simulink model "PV_SYSTEM_WITH_VARIOUS_MPPT"  (R2017a)
settings: Solver=ode45  StartTime=0.0  StopTime=2  RelTol=1e-3  EnableMultiTasking=on
undefined symbols (not defined in the file): dEgdT, EgRef, gcbh, k1, Rsh_array5pc, sigbuilder_block, sps_rtmsupport, Tref_K, Ts, VT_ref
libraries: powerlib x16, neural x15, simulink x4, spsPVarrayModel x3, powerlib_extras x2, fuzblock x1, powerlib_meascontrol x1
(part 6 of 6)

== system PV_SYSTEM_WITH_VARIOUS_MPPT/MATLAB//SIMULINK  BLOCK/      ==
  In1 : Inport
  In2 : Inport  Port=2
  Gain : Gain  Gain=100
  div1 : Product  Inputs=/*  RndMeth=Zero
  Out1 : Outport
  wires:
  Gain/1 -> Out1/1
  div1/1 -> Gain/1
  In2/1 -> div1/2
  In1/1 -> div1/1

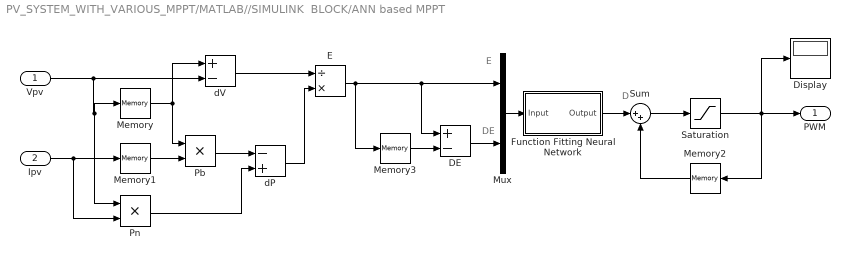
== system PV_SYSTEM_WITH_VARIOUS_MPPT/MATLAB//SIMULINK  BLOCK/ANN based MPPT ==
  note: E
  note: DE
  note: D
  Vpv : Inport
  Ipv : Inport  Port=2
  DE : Sum  Inputs=+-
  Display : Display
  E : Product  Inputs=/*
  Function Fitting Neural Network : Subsystem
      mask help: Function Fitting Neural Network
      mask Display: e = 0.06;c1 = [120 150 230]/255;c2 = ([120 150 230]+0)/383;c3 = ([120 150 230]+128)/383;patch([0 1 1 0],[0 0 1 1],c1);patch([0 1 1 1-e 1-e 0+e],[0 0 1 1-e 0+e 0+e],c2);patch([0 0 1 1-e 0+e 0+e],[0 1 1 1-e 1-e 0+e],c3);plot([0 1 1 0 0],[0 0 1 1 0]);fprintf('NNET');port_label('input',1,' Input');port_label('output',1,'Output ');
  Memory{,1..3} (4 alike) : Memory  InheritSampleTime=on
  Mux : Mux  Inputs=2
  Pb : Product
  Pn : Product
  Saturation : Saturate  UpperLimit=0.9  LowerLimit=0.1
  Sum : Sum  Inputs=|++
  dP : Sum  Inputs=-+
  dV : Sum  Inputs=+-
  PWM : Outport
  wires:
  Function Fitting Neural Network/1(Output) -> Sum/1
  Mux/1 -> Function Fitting Neural Network/1(Input)
  Sum/1 -> Saturation/1
  dV/1 -> E/1
  E/1 -> Memory3/1, Mux/1, DE/1
  dP/1 -> E/2
  Vpv/1 -> dV/2, Memory/1, Pn/1
  Saturation/1 -> Memory2/1, PWM/1, Display/1
  DE/1 -> Mux/2
  Memory3/1 -> DE/2
  Memory2/1 -> Sum/2
  Pn/1 -> dP/2
  Pb/1 -> dP/1
  Memory1/1 -> Pb/2
  Ipv/1 -> Memory1/1, Pn/2
  Memory/1 -> dV/1, Pb/1

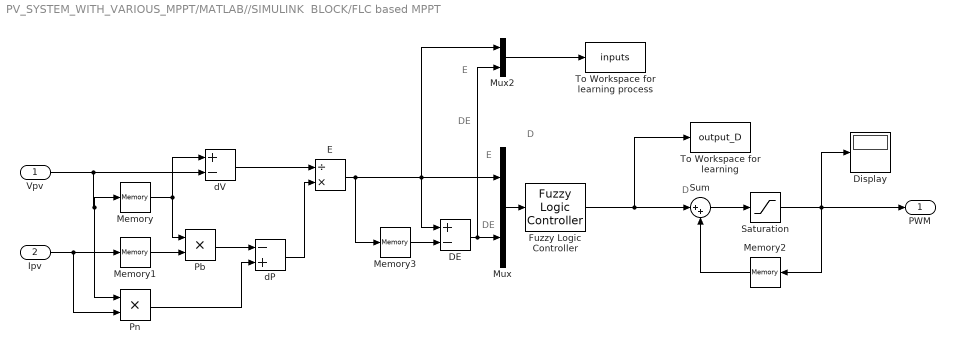
== system PV_SYSTEM_WITH_VARIOUS_MPPT/MATLAB//SIMULINK  BLOCK/FLC based MPPT ==
  note: DE
  note: D
  note: E
  note: D
  note: DE
  note: E
  Vpv : Inport
  Ipv : Inport  Port=2
  DE : Sum  Inputs=+-
  Display : Display
  E : Product  Inputs=/*
  Fuzzy Logic Controller : fuzblock/Fuzzy Logic  Controller  fis=mppt
  Memory{,1..3} (4 alike) : Memory  InheritSampleTime=on
  Mux : Mux  Inputs=2
  Mux2 : Mux  Inputs=2
  Pb : Product
  Pn : Product
  Saturation : Saturate  UpperLimit=0.9  LowerLimit=0.1
  Sum : Sum  Inputs=|++
  To Workspace for learning : ToWorkspace  VariableName=output_D  SampleTime=1e-6
      settings: MaxDataPoints=10000  Save2DSignal=2-D array (concatenate along first dimension)
  To Workspace for learning process : ToWorkspace  VariableName=inputs  SampleTime=1e-6
      settings: MaxDataPoints=100000  Save2DSignal=2-D array (concatenate along first dimension)
  dP : Sum  Inputs=-+
  dV : Sum  Inputs=+-
  PWM : Outport
  wires:
  Memory/1 -> Pb/1, dV/1
  Ipv/1 -> Pn/2, Memory1/1
  Memory1/1 -> Pb/2
  Pb/1 -> dP/1
  Pn/1 -> dP/2
  Memory2/1 -> Sum/2
  Memory3/1 -> DE/2
  DE/1 -> Mux/2, Mux2/2
  Saturation/1 -> Display/1, PWM/1, Memory2/1
  Vpv/1 -> Pn/1, Memory/1, dV/2
  dP/1 -> E/2
  E/1 -> DE/1, Mux/1, Mux2/1, Memory3/1
  dV/1 -> E/1
  Sum/1 -> Saturation/1
  Mux/1 -> Fuzzy Logic Controller/1
  Mux2/1 -> To Workspace for learning process/1
  Fuzzy Logic Controller/1 -> To Workspace for learning/1, Sum/1

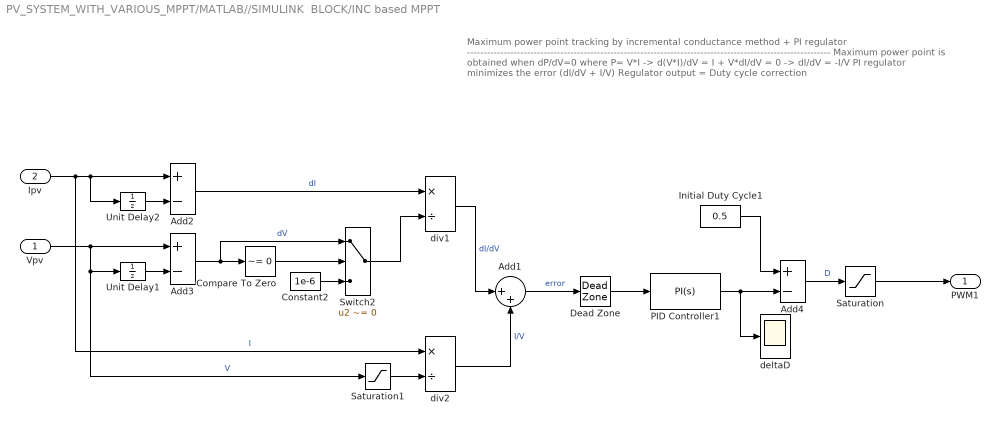
== system PV_SYSTEM_WITH_VARIOUS_MPPT/MATLAB//SIMULINK  BLOCK/INC based MPPT ==
  note: Maximum power point tracking by incremental conductance method + PI regulator
      | -------------------------------------------------------------------------------------------------------------
      | Maximum power point is obtained when dP/dV=0  where P= V*I
      | -> d(V*I)/dV = I + V*dI/dV = 0
      | -> dI/dV = -I/V
      | PI regulator minimizes the error (dI/dV + I/V)
      | Regulator output = Duty cycle correction
  Vpv : Inport
  Ipv : Inport  Port=2
  Add1 : Sum  Inputs=|++
  Add2 : Sum  Inputs=+-
  Add3 : Sum  Inputs=+-
  Add4 : Sum  Inputs=+-
  Compare To Zero : simulink/Logic and Bit Operations/Compare To Zero  relop=~=  OutDataTypeStr=uint8
  Constant2 : Constant  Value=1e-6
  Dead Zone : DeadZone  LowerValue=-0.02  UpperValue=+0.02  SaturateOnIntegerOverflow=on
  Initial Duty Cycle1 : Constant  Value=0.5
  PID Controller1 : simulink/Continuous/PID Controller  Controller=PI  TimeDomain=Continuous-time  SampleTime=-1  IntegratorMethod=Forward Euler  FilterMethod=Forward Euler  Form=Parallel  UseFilter=on  ControllerParametersSource=internal  P=8  I=20  D=0  N=100  InitialConditionSource=internal  InitialConditionForIntegrator=0  InitialConditionForFilter=0  ExternalReset=none  LimitOutput=on  UpperSaturationLimit=1  LowerSaturationLimit=-1  LinearizeAsGain=on  AntiWindupMode=none  Kb=1  TrackingMode=off  Kt=1  PParamMin=[]  PParamMax=[]  IParamMin=[]  IParamMax=[]  DParamMin=[]  DParamMax=[]  NParamMin=[]  NParamMax=[]  KbParamMin=[]  KbParamMax=[]  KtParamMin=[]  KtParamMax=[]  POutMin=[]  POutMax=[]  IOutMin=[]  IOutMax=[]  DOutMin=[]  DOutMax=[]  NOutMin=[]  NOutMax=[]  KbOutMin=[]  KbOutMax=[]  KtOutMin=[]  KtOutMax=[]  IntegratorOutMin=[]  IntegratorOutMax=[]  FilterOutMin=[]  FilterOutMax=[]  SumOutMin=[]  SumOutMax=[]  SumI1OutMin=[]  SumI1OutMax=[]  SumI2OutMin=[]  SumI2OutMax=[]  SumI3OutMin=[]  SumI3OutMax=[]  SumDOutMin=[]  SumDOutMax=[]  SaturationOutMin=[]  SaturationOutMax=[]  IntegratorContinuousStateAttributes=''  IntegratorStateMustResolveToSignalObject=off  IntegratorRTWStateStorageClass=Auto  FilterContinuousStateAttributes=''  FilterStateMustResolveToSignalObject=off  FilterRTWStateStorageClass=Auto  DifferentiatorICPrevScaledInput=0  DifferentiatorOutMin=[]  DifferentiatorOutMax=[]  InitialConditionSetting=State (most efficient)
  Saturation : Saturate  UpperLimit=1  LowerLimit=0
  Saturation1 : Saturate  UpperLimit=inf  LowerLimit=eps
  Switch2 : Switch  Criteria=u2 ~= 0
  Unit Delay1 : UnitDelay  SampleTime=Ts
  Unit Delay2 : UnitDelay  SampleTime=Ts
  deltaD : Scope
  div1 : Product  Inputs=*/  RndMeth=Zero
  div2 : Product  Inputs=*/  RndMeth=Zero
  PWM1 : Outport
  wires:
  Add4/1 -> Saturation/1  "D"
  PID Controller1/1 -> deltaD/1, Add4/2
  Initial Duty Cycle1/1 -> Add4/1
  Add3/1 -> Compare To Zero/1, Switch2/1  "dV"
  div2/1 -> Add1/2  "I/V"
  Saturation1/1 -> div2/2
  Unit Delay1/1 -> Add3/2
  Add2/1 -> div1/1  "dI"
  Switch2/1 -> div1/2
  Unit Delay2/1 -> Add2/2
  Ipv/1 -> Unit Delay2/1, Add2/1, div2/1  "I"
  div1/1 -> Add1/1  "dI/dV"
  Compare To Zero/1 -> Switch2/2
  Constant2/1 -> Switch2/3
  Vpv/1 -> Add3/1, Saturation1/1, Unit Delay1/1  "V"
  Add1/1 -> Dead Zone/1  "error"
  Dead Zone/1 -> PID Controller1/1
  Saturation/1 -> PWM1/1

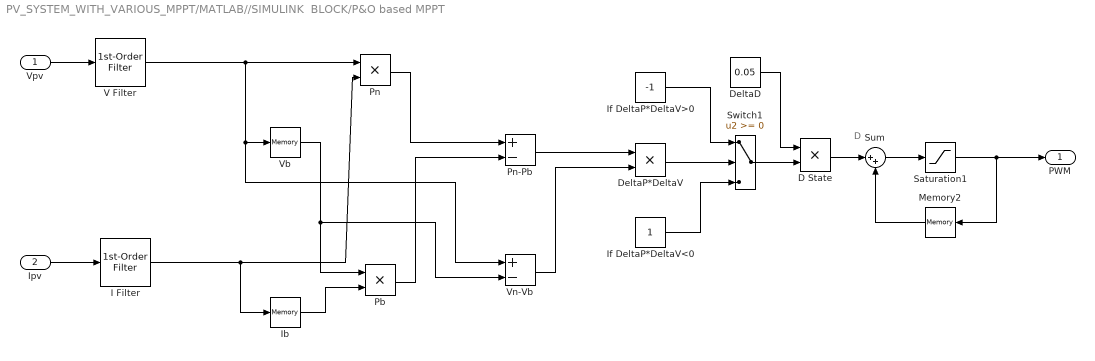
== system PV_SYSTEM_WITH_VARIOUS_MPPT/MATLAB//SIMULINK  BLOCK/P&O based MPPT ==
  note: D
  Vpv : Inport
  Ipv : Inport  Port=2
  D State : Product  RndMeth=Zero
  DeltaD : Constant  Value=0.05
  DeltaP*DeltaV : Product  RndMeth=Zero
  I Filter : powerlib_extras/Control  Blocks/1st-Order  Filter  FilterType=Lowpass  Tc=1e-3  Initialize=off  Vac_Init=[0.8 -25 60]  Vdc_Init=-0.4  PlotResponse=off  param1=[1 500 1]
  Ib : Memory  InheritSampleTime=on  LinearizeAsDelay=on
  If DeltaP*DeltaV<0 : Constant
  If DeltaP*DeltaV>0 : Constant  Value=-1
  Memory2 : Memory  InheritSampleTime=on
  Pb : Product  RndMeth=Zero
  Pn : Product  RndMeth=Zero
  Pn-Pb : Sum  Inputs=+-
  Saturation1 : Saturate  UpperLimit=0.9  LowerLimit=0.1
  Sum : Sum  Inputs=|++
  Switch1 : Switch
  V Filter : powerlib_extras/Control  Blocks/1st-Order  Filter  FilterType=Lowpass  Tc=1e-3  Initialize=off  Vac_Init=[0.8 -25 60]  Vdc_Init=-0.4  PlotResponse=off  param1=[1 500 1]
  Vb : Memory  InheritSampleTime=on  LinearizeAsDelay=on
  Vn-Vb : Sum  Inputs=+-
  PWM : Outport
  wires:
  Ipv/1 -> I Filter/1
  If DeltaP*DeltaV<0/1 -> Switch1/3
  Pn/1 -> Pn-Pb/1
  V Filter/1 -> Vn-Vb/1, Vb/1, Pn/1
  Ib/1 -> Pb/2
  DeltaP*DeltaV/1 -> Switch1/2
  Vb/1 -> Vn-Vb/2, Pb/1
  If DeltaP*DeltaV>0/1 -> Switch1/1
  Pn-Pb/1 -> DeltaP*DeltaV/1
  Vn-Vb/1 -> DeltaP*DeltaV/2
  I Filter/1 -> Pn/2, Ib/1
  Vpv/1 -> V Filter/1
  Pb/1 -> Pn-Pb/2
  Switch1/1 -> D State/2
  DeltaD/1 -> D State/1
  D State/1 -> Sum/1
  Sum/1 -> Saturation1/1
  Memory2/1 -> Sum/2
  Saturation1/1 -> PWM/1, Memory2/1

== system PV_SYSTEM_WITH_VARIOUS_MPPT/MATLAB//SIMULINK  BLOCK/X-Y Plotter ==
  x : Inport
  y : Inport  Port=2
  Setting : Constant  Value=[N xmin xmax ymin ymax]
  X-Y Animated Plotter : MATLAB Function  TreatAsAtomicUnit=on  SystemSampleTime=tsam
  wires:
  Setting/1 -> X-Y Animated Plotter/3(set)
  y/1 -> X-Y Animated Plotter/2(y)
  x/1 -> X-Y Animated Plotter/1(x)

== system PV_SYSTEM_WITH_VARIOUS_MPPT/MATLAB//SIMULINK  BLOCK/	PV panels of LREA laboratory /Irradiance  ==
  Demux : Demux  Tag=STV Demux  Outputs=2
  FromWs : FromWorkspace  Tag=STV FromWs  VariableName=tuvar  SampleTime=0
      SigBuilderData=|
      | common.afterFinalStr = 'Extrapolate'
      | common.sampleTime = '0'
      | dataSet(1).timeRange = [0 2]
      | dataSet(1).name = 'Constant Irradiance'
      | dataSet(2).timeRange = [0 2]
      | dataSet(2).name = 'Step Irradiance'
      | dataSet(3).timeRange = [0 1]
      | dataSet(3).name = 'Ramp-up/down Irradiance'
      | sbobj.Groups(1).Name = 'Constant Irradiance'
      | sbobj.Groups(1).Signals(1).Name = 'Ir'
      | sbobj.Groups(1).Signals(1).XData = [0 2]
      | sbobj.Groups(1).Signals(1).YData = [1000 1000]
      | sbobj.Groups(1).Signals(2).Name = 'Temp'
      | sbobj.Groups(1).Signals(2).XData = [0 1 1 2]
      | sbobj.Groups(1).Signals(2).YData = [0 0 1 1]
      | sbobj.Groups(1).TimeRange = [0 2]
      | sbobj.Groups(2).Name = 'Step Irradiance'
      | sbobj.Groups(2).Signals(1).Name = 'Ir'
      | sbobj.Groups(2).Signals(1).XData = [0 0.252 0.252 2]
      | sbobj.Groups(2).Signals(1).YData = [600 600 1000 1000]
      | sbobj.Groups(2).Signals(2).Name = 'Temp'
      | sbobj.Groups(2).Signals(2).XData = [0 1 1 2]
      | sbobj.Groups(2).Signals(2).YData = [0 0 1 1]
      | sbobj.Groups(2).TimeRange = [0 2]
      | sbobj.Groups(3).Name = 'Ramp-up/down Irradiance'
      | sbobj.Groups(3).Signals(1).Name = 'Ir'
      | sbobj.Groups(3).Signals(1).XData = [0 0.3 0.3 0.4 0.4 0.5 0.5 1]
      | sbobj.Groups(3).Signals(1).YData = [1000 1000 800 795 600 600 400 395]
      | sbobj.Groups(3).Signals(2).Name = 'Temp'
      | sbobj.Groups(3).Signals(2).XData = [0 1]
      | sbobj.Groups(3).Signals(2).YData = [25 25]
      | sbobj.Groups(3).TimeRange = [0 1]
  Ir : Outport  Tag=STV Outport
  Temp : Outport  Tag=STV Outport  Port=2
  wires:
  Demux/1 -> Ir/1
  FromWs/1 -> Demux/1
  Demux/2 -> Temp/1

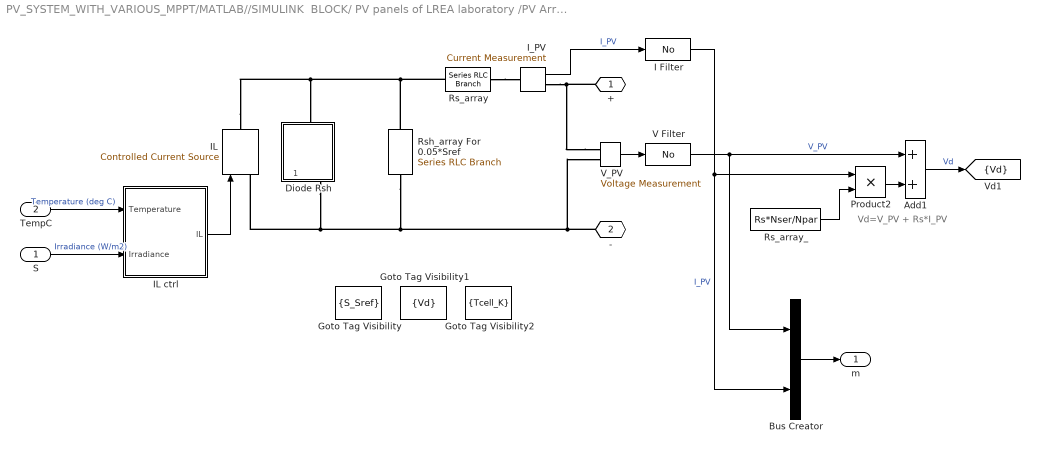
== system PV_SYSTEM_WITH_VARIOUS_MPPT/MATLAB//SIMULINK  BLOCK/	PV panels of LREA laboratory /PV Array ==
  note: Vd=V_PV + Rs*I_PV
  S : Inport
  TempC : Inport  Port=2
  Add1 : Sum
  Bus Creator : BusCreator  Inputs=2
  Diode Rsh : Subsystem
      mask Display:
      | plot(-75,-50,100,150, [-15 -15 43 -15 -15 -75],[50 8 50 92 50 50], ...
      |     [43 43],[8 94],[100 43], [50 50])
  Goto Tag Visibility : GotoTagVisibility  GotoTag=S_Sref
  Goto Tag Visibility1 : GotoTagVisibility  GotoTag=Vd
  Goto Tag Visibility2 : GotoTagVisibility  GotoTag=Tcell_K
  I Filter : spsPVarrayModel/No  VariantControl=Variant1
  IL : powerlib/Electrical Sources/Controlled Current Source  Initialize=on  Source_Type=AC  Amplitude=0  Phase=0  Frequency=0  Measurements=None
  IL ctrl : Subsystem
  I_PV : powerlib/Measurements/Current Measurement  PhasorSimulation=off  OutputType=Complex  PSBequivalent=0
  Product2 : Product  Inputs=**  RndMeth=Zero
  Rs_array : powerlib/Elements/Series RLC Branch  LConnTagsString=__new0  RConnTagsString=__new0  BranchType=R  Resistance=Rs*Nser/Npar  Inductance=1e-3  SetiL0=off  InitialCurrent=0  Capacitance=1e-6  Setx0=off  InitialVoltage=0  Measurements=None
  Rs_array_ : Constant  Value=Rs*Nser/Npar
  Rsh_array For 0.05*Sref : powerlib/Elements/Series RLC Branch  LConnTagsString=__new0  RConnTagsString=__new0  BranchType=R  Resistance=Rsh_array5pc  Inductance=1e-3  SetiL0=off  InitialCurrent=0  Capacitance=1e-6  Setx0=off  InitialVoltage=0  Measurements=None
  V Filter : spsPVarrayModel/No  VariantControl=Variant1
  V_PV : powerlib/Measurements/Voltage Measurement  PhasorSimulation=off  OutputType=Complex  PSBequivalent=0
  + : PMIOPort  Port=1  Side=Right
  - : PMIOPort  Port=2  Side=Right
  m : Outport
  tag scope: Vd=scoped
  wires:
  V Filter/1 -> Add1/1, Bus Creator/1  "V_PV"
  I Filter/1 -> Product2/1, Bus Creator/2  "I_PV"
  V_PV/1 -> V Filter/1
  IL ctrl/1(IL) -> IL/1
  Bus Creator/1 -> m/1
  Rs_array_/1 -> Product2/2
  Product2/1 -> Add1/2
  I_PV/1 -> I Filter/1  "I_PV"
  Add1/1 -> [Vd]  "Vd"
  S/1 -> IL ctrl/2(Irradiance)  "Irradiance (W/m2)"
  TempC/1 -> IL ctrl/1(Temperature)  "Temperature (deg C)"
  connections:
  Rs_array/RConn1 -- I_PV/LConn1
  IL/LConn1 -- Diode Rsh/RConn1 -- Rsh_array For 0.05*Sref/RConn1 -- -/RConn1 -- V_PV/LConn2
  IL/RConn1 -- Rsh_array For 0.05*Sref/LConn1 -- Rs_array/LConn1 -- Diode Rsh/LConn1
  V_PV/LConn1 -- I_PV/RConn1 -- +/RConn1

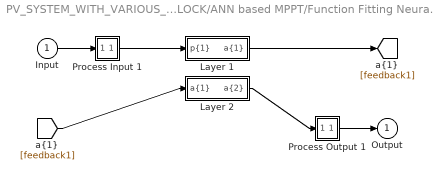
== system PV_SYSTEM_WITH_VARIOUS_MPPT/MATLAB//SIMULINK  BLOCK/ANN based MPPT/Function Fitting Neural Network ==
  Input : Inport  PortDimensions=2
      mask Display: e = 0.06;c1 = [120 230 180]/255;c2 = ([120 230 180]+0)/(256+128);c3 = ([120 230 180]+128)/(256+128);patch([0 1 1 0],[0 0 1 1],c1);patch([0 1 1 1-e 1-e 0+e],[0 0 1 1-e 0+e 0+e],c2);patch([0 0 1 1-e 0+e 0+e],[0 1 1 1-e 1-e 0+e],c3);plot([0 1 1 0 0],[0 0 1 1 0]);
  Layer 1 : Subsystem
      mask Display: e = 0.06;c1 = [120 150 230]/255;c2 = ([120 150 230]+0)/383;c3 = ([120 150 230]+128)/383;patch([0 1 1 0],[0 0 1 1],c1);patch([0 1 1 1-e 1-e 0+e],[0 0 1 1-e 0+e 0+e],c2);patch([0 0 1 1-e 0+e 0+e],[0 1 1 1-e 1-e 0+e],c3);plot([0 1 1 0 0],[0 0 1 1 0]);
  Layer 2 : Subsystem
      mask Display: e = 0.06;c1 = [120 150 230]/255;c2 = ([120 150 230]+0)/383;c3 = ([120 150 230]+128)/383;patch([0 1 1 0],[0 0 1 1],c1);patch([0 1 1 1-e 1-e 0+e],[0 0 1 1-e 0+e 0+e],c2);patch([0 0 1 1-e 0+e 0+e],[0 1 1 1-e 1-e 0+e],c3);plot([0 1 1 0 0],[0 0 1 1 0]);
  Process Input 1 : Subsystem
      mask Display: e = 0.06;c1 = [120 150 230]/255;c2 = ([120 150 230]+0)/383;c3 = ([120 150 230]+128)/383;patch([0 1 1 0],[0 0 1 1],c1);patch([0 1 1 1-e 1-e 0+e],[0 0 1 1-e 0+e 0+e],c2);patch([0 0 1 1-e 0+e 0+e],[0 1 1 1-e 1-e 0+e],c3);plot([0 1 1 0 0],[0 0 1 1 0]);
  Process Output 1 : Subsystem
      mask Display: e = 0.06;c1 = [120 150 230]/255;c2 = ([120 150 230]+0)/383;c3 = ([120 150 230]+128)/383;patch([0 1 1 0],[0 0 1 1],c1);patch([0 1 1 1-e 1-e 0+e],[0 0 1 1-e 0+e 0+e],c2);patch([0 0 1 1-e 0+e 0+e],[0 1 1 1-e 1-e 0+e],c3);plot([0 1 1 0 0],[0 0 1 1 0]);
  Output : Outport  InitialOutput=0
      mask Display: e = 0.06;c1 = [120 230 180]/255;c2 = ([120 230 180]+0)/(256+128);c3 = ([120 230 180]+128)/(256+128);patch([0 1 1 0],[0 0 1 1],c1);patch([0 1 1 1-e 1-e 0+e],[0 0 1 1-e 0+e 0+e],c2);patch([0 0 1 1-e 0+e 0+e],[0 1 1 1-e 1-e 0+e],c3);plot([0 1 1 0 0],[0 0 1 1 0]);
  wires:
  Layer 2/1("a{2}") -> Process Output 1/1(a)
  [feedback1] -> Layer 2/1("a{1} ")
  Layer 1/1("a{1}") -> [feedback1]
  Process Input 1/1(p) -> Layer 1/1("p{1}")
  Process Output 1/1(y) -> Output/1
  Input/1 -> Process Input 1/1(x)

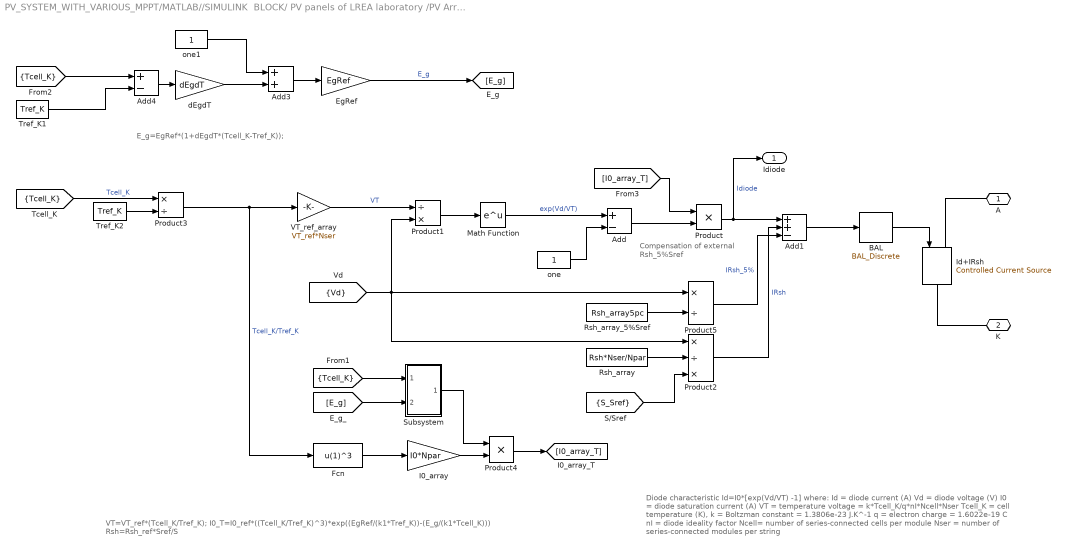
== system PV_SYSTEM_WITH_VARIOUS_MPPT/MATLAB//SIMULINK  BLOCK/	PV panels of LREA laboratory /PV Array/Diode Rsh ==
  note: Compensation of
      | external Rsh_5%Sref
  note: Diode characteristic
      |    Id=I0*[exp(Vd/VT) -1]
      |
      | where:
      |      Id = diode current (A)
      |      Vd = diode voltage (V)
      |      I0 = diode saturation current (A)
      |      VT = temperature voltage = k*Tcell_K/q*nI*Ncell*Nser
      | Tcell_K = cell temperature (K),
      |       k = Boltzman constant = 1.3806e-23 J.K^-1
      |       q = electron charge = 1.6022e-19 C
      |      nI = diode ideality factor
      |    Ncell= number of series-connected cells per module
      |    Nser = number of series-connected modules per string
  note: VT=VT_ref*(Tcell_K/Tref_K);
      | I0_T=I0_ref*((Tcell_K/Tref_K)^3)*exp((EgRef/(k1*Tref_K))-(E_g/(k1*Tcell_K)))
      | Rsh=Rsh_ref*Sref/S
  note: E_g=EgRef*(1+dEgdT*(Tcell_K-Tref_K));
  Add : Sum  Inputs=+-
  Add1 : Sum  Inputs=++-
  Add3 : Sum
  Add4 : Sum  Inputs=+-
  BAL : spsPVarrayModel/BAL_Discrete  VariantControl=NoBAL
  EgRef : Gain  Gain=EgRef
  Fcn : Fcn  Expr=u(1)^3
  I0_array : Gain  Gain=I0*Npar
  Id+IRsh : powerlib/Electrical Sources/Controlled Current Source  Initialize=on  Source_Type=AC  Amplitude=0  Phase=0  Frequency=0  Measurements=None
  Math Function : Math  SaturateOnIntegerOverflow=on
  Product : Product  RndMeth=Zero
  Product1 : Product  Inputs=/*  RndMeth=Zero
  Product2 : Product  Inputs=*/*  RndMeth=Zero
  Product3 : Product  Inputs=*/  RndMeth=Zero
  Product4 : Product  Inputs=**  RndMeth=Zero
  Product5 : Product  Inputs=*/  RndMeth=Zero
  Rsh_array : Constant  Value=Rsh*Nser/Npar
  Rsh_array_5%Sref : Constant  Value=Rsh_array5pc
  Subsystem : Subsystem
  Tref_K1 : Constant  Value=Tref_K
  Tref_K2 : Constant  Value=Tref_K
  VT_ref_array : Gain  Gain=VT_ref*Nser
  dEgdT : Gain  Gain=dEgdT
  one : Constant
  one1 : Constant
  A : PMIOPort  Port=1  Side=Left
  K : PMIOPort  Port=2  Side=Right
  Idiode : Outport
  wires:
  BAL/1 -> Id+IRsh/1
  Add1/1 -> BAL/1
  Product5/1 -> Add1/3  "IRsh_5%"
  Rsh_array_5%Sref/1 -> Product5/2
  Math Function/1 -> Add/1  "exp(Vd/VT)"
  Product2/1 -> Add1/2  "IRsh"
  Product/1 -> Add1/1, Idiode/1  "Idiode"
  Product1/1 -> Math Function/1
  one/1 -> Add/2
  Rsh_array/1 -> Product2/2
  [Tcell_K] -> Product3/1  "Tcell_K"
  Product3/1 -> VT_ref_array/1, Fcn/1  "Tcell_K/Tref_K"
  one1/1 -> Add3/1
  Add4/1 -> dEgdT/1
  dEgdT/1 -> Add3/2
  Add3/1 -> EgRef/1
  EgRef/1 -> [E_g]  "E_g"
  I0_array/1 -> Product4/2
  Fcn/1 -> I0_array/1
  [Tcell_K] -> Add4/1
  Tref_K1/1 -> Add4/2
  Subsystem/1(exp) -> Product4/1
  [Tcell_K] -> Subsystem/1(Tcell_K)
  [E_g] -> Subsystem/2(E_g)
  Tref_K2/1 -> Product3/2
  Product4/1 -> [I0_array_T]
  Add/1 -> Product/2
  VT_ref_array/1 -> Product1/1  "VT"
  [I0_array_T] -> Product/1
  [S_Sref] -> Product2/3
  [Vd] -> Product5/1, Product2/1, Product1/2
  connections:
  Id+IRsh/RConn1 -- K/RConn1
  A/RConn1 -- Id+IRsh/LConn1

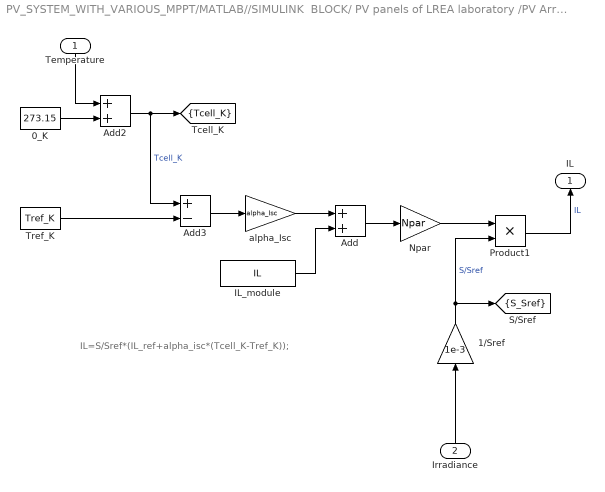
== system PV_SYSTEM_WITH_VARIOUS_MPPT/MATLAB//SIMULINK  BLOCK/	PV panels of LREA laboratory /PV Array/IL ctrl ==
  note: IL=S/Sref*(IL_ref+alpha_isc*(Tcell_K-Tref_K));
  Temperature : Inport
  Irradiance : Inport  Port=2
  0_K : Constant  Value=273.15
  1/Sref : Gain  Gain=1e-3
  Add : Sum
  Add2 : Sum
  Add3 : Sum  Inputs=+-
  IL_module : Constant  Value=IL
  Npar : Gain  Gain=Npar
  Product1 : Product  Inputs=**  RndMeth=Zero
  Tref_K : Constant  Value=Tref_K
  alpha_Isc : Gain  Gain=alpha_Isc
  IL : Outport
  tag scope: S_Sref=scoped, Tcell_K=scoped
  wires:
  Temperature/1 -> Add2/1
  Irradiance/1 -> 1/Sref/1
  alpha_Isc/1 -> Add/1
  Add3/1 -> alpha_Isc/1
  Tref_K/1 -> Add3/2
  Product1/1 -> IL/1  "IL"
  IL_module/1 -> Add/2
  0_K/1 -> Add2/2
  Add/1 -> Npar/1
  Add2/1 -> Add3/1, [Tcell_K]  "Tcell_K"
  Npar/1 -> Product1/1
  1/Sref/1 -> Product1/2, [S_Sref]  "S/Sref"

== system PV_SYSTEM_WITH_VARIOUS_MPPT/MATLAB//SIMULINK  BLOCK/ANN based MPPT/Function Fitting Neural Network/Layer 1 ==
  "p{1}" : Inport  PortDimensions=2
      mask Display: e = 0.06;c1 = [120 230 180]/255;c2 = ([120 230 180]+0)/(256+128);c3 = ([120 230 180]+128)/(256+128);patch([0 1 1 0],[0 0 1 1],c1);patch([0 1 1 1-e 1-e 0+e],[0 0 1 1-e 0+e 0+e],c2);patch([0 0 1 1-e 0+e 0+e],[0 1 1 1-e 1-e 0+e],c3);plot([0 1 1 0 0],[0 0 1 1 0]);
  Delays 1 : Subsystem
      mask Display: e = 0.06;c1 = [120 150 230]/255;c2 = ([120 150 230]+0)/383;c3 = ([120 150 230]+128)/383;patch([0 1 1 0],[0 0 1 1],c1);patch([0 1 1 1-e 1-e 0+e],[0 0 1 1-e 0+e 0+e],c2);patch([0 0 1 1-e 0+e 0+e],[0 1 1 1-e 1-e 0+e],c3);plot([0 1 1 0 0],[0 0 1 1 0]);disp('0');
  "IW{1,1}" : Subsystem
      mask Display: e = 0.06;c1 = [120 150 230]/255;c2 = ([120 150 230]+0)/383;c3 = ([120 150 230]+128)/383;patch([0 1 1 0],[0 0 1 1],c1);patch([0 1 1 1-e 1-e 0+e],[0 0 1 1-e 0+e 0+e],c2);patch([0 0 1 1-e 0+e 0+e],[0 1 1 1-e 1-e 0+e],c3);plot([0 1 1 0 0],[0 0 1 1 0]);disp('W');
  "b{1}" : Constant  Value=[4.2498450600033646;-3.5459947004323884;-2.8437309415280434;1.9169166361344252;-0.42994895301969316;-0.41524374608432507;1.5012029363474229;2.4596143283853529;3.4420068184056949;4.4215289791863901]
      mask Display: e = 0.06;c1 = [120 150 230]/255;c2 = ([120 150 230]+0)/383;c3 = ([120 150 230]+128)/383;patch([0 1 1 0],[0 0 1 1],c1);patch([0 1 1 1-e 1-e 0+e],[0 0 1 1-e 0+e 0+e],c2);patch([0 0 1 1-e 0+e 0+e],[0 1 1 1-e 1-e 0+e],c3);plot([0 1 1 0 0],[0 0 1 1 0]);disp('b');
  netsum : Sum  Inputs=2  SaturateOnIntegerOverflow=on  InputSameDT=on  OutDataTypeStr=Inherit: Same as first input
      mask Display: e = 0.06;c1 = [120 150 230]/255;c2 = ([120 150 230]+0)/383;c3 = ([120 150 230]+128)/383;patch([0 1 1 0],[0 0 1 1],c1);patch([0 1 1 1-e 1-e 0+e],[0 0 1 1-e 0+e 0+e],c2);patch([0 0 1 1-e 0+e 0+e],[0 1 1 1-e 1-e 0+e],c3);plot([0 1 1 0 0],[0 0 1 1 0]);disp('+');
  tansig : neural/Transfer Functions/tansig
  "a{1}" : Outport  InitialOutput=[0;0;0;0;0;0;0;0;0;0]
      mask Display: e = 0.06;c1 = [120 230 180]/255;c2 = ([120 230 180]+0)/(256+128);c3 = ([120 230 180]+128)/(256+128);patch([0 1 1 0],[0 0 1 1],c1);patch([0 1 1 1-e 1-e 0+e],[0 0 1 1-e 0+e 0+e],c2);patch([0 0 1 1-e 0+e 0+e],[0 1 1 1-e 1-e 0+e],c3);plot([0 1 1 0 0],[0 0 1 1 0]);
  wires:
  tansig/1 -> "a{1}"/1
  netsum/1 -> tansig/1
  "b{1}"/1 -> netsum/2
  "IW{1,1}"/1("iz{1,1}") -> netsum/1
  Delays 1/1("pd{1,1}") -> "IW{1,1}"/1("pd{1,1}")
  "p{1}"/1 -> Delays 1/1("p{1}")

== system PV_SYSTEM_WITH_VARIOUS_MPPT/MATLAB//SIMULINK  BLOCK/ANN based MPPT/Function Fitting Neural Network/Layer 2 ==
  "a{1} " : Inport  PortDimensions=10
      mask Display: e = 0.06;c1 = [120 230 180]/255;c2 = ([120 230 180]+0)/(256+128);c3 = ([120 230 180]+128)/(256+128);patch([0 1 1 0],[0 0 1 1],c1);patch([0 1 1 1-e 1-e 0+e],[0 0 1 1-e 0+e 0+e],c2);patch([0 0 1 1-e 0+e 0+e],[0 1 1 1-e 1-e 0+e],c3);plot([0 1 1 0 0],[0 0 1 1 0]);
  Delays 1 : Subsystem
      mask Display: e = 0.06;c1 = [120 150 230]/255;c2 = ([120 150 230]+0)/383;c3 = ([120 150 230]+128)/383;patch([0 1 1 0],[0 0 1 1],c1);patch([0 1 1 1-e 1-e 0+e],[0 0 1 1-e 0+e 0+e],c2);patch([0 0 1 1-e 0+e 0+e],[0 1 1 1-e 1-e 0+e],c3);plot([0 1 1 0 0],[0 0 1 1 0]);disp('0');
  "LW{2,1}" : Subsystem
      mask Display: e = 0.06;c1 = [120 150 230]/255;c2 = ([120 150 230]+0)/383;c3 = ([120 150 230]+128)/383;patch([0 1 1 0],[0 0 1 1],c1);patch([0 1 1 1-e 1-e 0+e],[0 0 1 1-e 0+e 0+e],c2);patch([0 0 1 1-e 0+e 0+e],[0 1 1 1-e 1-e 0+e],c3);plot([0 1 1 0 0],[0 0 1 1 0]);disp('W');
  "b{2}" : Constant  Value=1.5159961723017756
      mask Display: e = 0.06;c1 = [120 150 230]/255;c2 = ([120 150 230]+0)/383;c3 = ([120 150 230]+128)/383;patch([0 1 1 0],[0 0 1 1],c1);patch([0 1 1 1-e 1-e 0+e],[0 0 1 1-e 0+e 0+e],c2);patch([0 0 1 1-e 0+e 0+e],[0 1 1 1-e 1-e 0+e],c3);plot([0 1 1 0 0],[0 0 1 1 0]);disp('b');
  netsum : Sum  Inputs=2  SaturateOnIntegerOverflow=on  InputSameDT=on  OutDataTypeStr=Inherit: Same as first input
      mask Display: e = 0.06;c1 = [120 150 230]/255;c2 = ([120 150 230]+0)/383;c3 = ([120 150 230]+128)/383;patch([0 1 1 0],[0 0 1 1],c1);patch([0 1 1 1-e 1-e 0+e],[0 0 1 1-e 0+e 0+e],c2);patch([0 0 1 1-e 0+e 0+e],[0 1 1 1-e 1-e 0+e],c3);plot([0 1 1 0 0],[0 0 1 1 0]);disp('+');
  purelin : neural/Transfer Functions/purelin
  "a{2}" : Outport  InitialOutput=0
      mask Display: e = 0.06;c1 = [120 230 180]/255;c2 = ([120 230 180]+0)/(256+128);c3 = ([120 230 180]+128)/(256+128);patch([0 1 1 0],[0 0 1 1],c1);patch([0 1 1 1-e 1-e 0+e],[0 0 1 1-e 0+e 0+e],c2);patch([0 0 1 1-e 0+e 0+e],[0 1 1 1-e 1-e 0+e],c3);plot([0 1 1 0 0],[0 0 1 1 0]);
  wires:
  purelin/1 -> "a{2}"/1
  netsum/1 -> purelin/1
  "b{2}"/1 -> netsum/2
  "LW{2,1}"/1("lz{2,1}") -> netsum/1
  Delays 1/1("pd{2,1}") -> "LW{2,1}"/1("ad{2,1}")
  "a{1} "/1 -> Delays 1/1("p{2}")

== system PV_SYSTEM_WITH_VARIOUS_MPPT/MATLAB//SIMULINK  BLOCK/ANN based MPPT/Function Fitting Neural Network/Process Input 1 ==
  x : Inport  PortDimensions=2
      mask Display: e = 0.06;c1 = [120 230 180]/255;c2 = ([120 230 180]+0)/(256+128);c3 = ([120 230 180]+128)/(256+128);patch([0 1 1 0],[0 0 1 1],c1);patch([0 1 1 1-e 1-e 0+e],[0 0 1 1-e 0+e 0+e],c2);patch([0 0 1 1-e 0+e 0+e],[0 1 1 1-e 1-e 0+e],c3);plot([0 1 1 0 0],[0 0 1 1 0]);
  mapminmax : neural/Processing Functions/mapminmax  xmin=[-94.016320043316156;-101.91504684015196]  xmax=[7.8987267968357999;90.85267225948256]  ymin=-1  ymax=1
  p : Outport  PortDimensions=2
      mask Display: e = 0.06;c1 = [120 230 180]/255;c2 = ([120 230 180]+0)/(256+128);c3 = ([120 230 180]+128)/(256+128);patch([0 1 1 0],[0 0 1 1],c1);patch([0 1 1 1-e 1-e 0+e],[0 0 1 1-e 0+e 0+e],c2);patch([0 0 1 1-e 0+e 0+e],[0 1 1 1-e 1-e 0+e],c3);plot([0 1 1 0 0],[0 0 1 1 0]);
  wires:
  mapminmax/1 -> p/1
  x/1 -> mapminmax/1

== system PV_SYSTEM_WITH_VARIOUS_MPPT/MATLAB//SIMULINK  BLOCK/ANN based MPPT/Function Fitting Neural Network/Process Output 1 ==
  a : Inport  PortDimensions=1
      mask Display: e = 0.06;c1 = [120 230 180]/255;c2 = ([120 230 180]+0)/(256+128);c3 = ([120 230 180]+128)/(256+128);patch([0 1 1 0],[0 0 1 1],c1);patch([0 1 1 1-e 1-e 0+e],[0 0 1 1-e 0+e 0+e],c2);patch([0 0 1 1-e 0+e 0+e],[0 1 1 1-e 1-e 0+e],c3);plot([0 1 1 0 0],[0 0 1 1 0]);
  mapminmax_reverse : neural/Processing Functions/mapminmax_reverse  xmin=-0.033148830521161396  xmax=0.087011804847006088  ymin=-1  ymax=1
  y : Outport  PortDimensions=1
      mask Display: e = 0.06;c1 = [120 230 180]/255;c2 = ([120 230 180]+0)/(256+128);c3 = ([120 230 180]+128)/(256+128);patch([0 1 1 0],[0 0 1 1],c1);patch([0 1 1 1-e 1-e 0+e],[0 0 1 1-e 0+e 0+e],c2);patch([0 0 1 1-e 0+e 0+e],[0 1 1 1-e 1-e 0+e],c3);plot([0 1 1 0 0],[0 0 1 1 0]);
  wires:
  mapminmax_reverse/1 -> y/1
  a/1 -> mapminmax_reverse/1

== system PV_SYSTEM_WITH_VARIOUS_MPPT/MATLAB//SIMULINK  BLOCK/	PV panels of LREA laboratory /PV Array/Diode Rsh/Subsystem ==
  note: exp((EgRef/(k1*Tref_K))-(E_g/(k1*Tcell_K)))
  Tcell_K : Inport
  E_g : Inport  Port=2
  Add : Sum  Inputs=+-
  EgRef : Constant  Value=EgRef/(k1*Tref_K)
  Math Function : Math  SaturateOnIntegerOverflow=on
  Product : Product  Inputs=*/
  k1 : Gain  Gain=k1
  exp : Outport
  wires:
  EgRef/1 -> Add/1
  E_g/1 -> Product/1
  Tcell_K/1 -> k1/1
  k1/1 -> Product/2
  Product/1 -> Add/2
  Add/1 -> Math Function/1
  Math Function/1 -> exp/1

== system PV_SYSTEM_WITH_VARIOUS_MPPT/MATLAB//SIMULINK  BLOCK/ANN based MPPT/Function Fitting Neural Network/Layer 1/Delays 1 ==
  "p{1}" : Inport  PortDimensions=2
      mask Display: e = 0.06;c1 = [120 230 180]/255;c2 = ([120 230 180]+0)/(256+128);c3 = ([120 230 180]+128)/(256+128);patch([0 1 1 0],[0 0 1 1],c1);patch([0 1 1 1-e 1-e 0+e],[0 0 1 1-e 0+e 0+e],c2);patch([0 0 1 1-e 0+e 0+e],[0 1 1 1-e 1-e 0+e],c3);plot([0 1 1 0 0],[0 0 1 1 0]);
  mux : Mux  Inputs=1
      mask Display: e = 0.06;c1 = [120 150 230]/255;c2 = ([120 150 230]+0)/383;c3 = ([120 150 230]+128)/383;patch([0 1 1 0],[0 0 1 1],c1);patch([0 1 1 1-e 1-e 0+e],[0 0 1 1-e 0+e 0+e],c2);patch([0 0 1 1-e 0+e 0+e],[0 1 1 1-e 1-e 0+e],c3);plot([0 1 1 0 0],[0 0 1 1 0]);disp('Mux')
  "pd{1,1}" : Outport
      mask Display: e = 0.06;c1 = [120 230 180]/255;c2 = ([120 230 180]+0)/(256+128);c3 = ([120 230 180]+128)/(256+128);patch([0 1 1 0],[0 0 1 1],c1);patch([0 1 1 1-e 1-e 0+e],[0 0 1 1-e 0+e 0+e],c2);patch([0 0 1 1-e 0+e 0+e],[0 1 1 1-e 1-e 0+e],c3);plot([0 1 1 0 0],[0 0 1 1 0]);
  wires:
  mux/1 -> "pd{1,1}"/1
  "p{1}"/1 -> mux/1

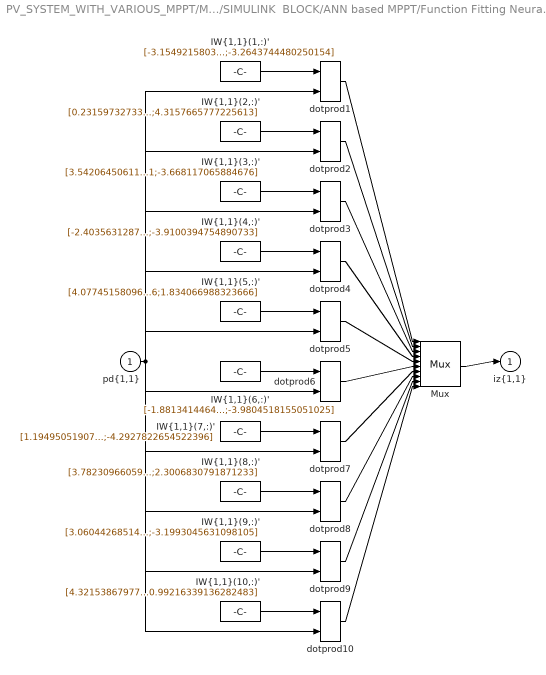
== system PV_SYSTEM_WITH_VARIOUS_MPPT/MATLAB//SIMULINK  BLOCK/ANN based MPPT/Function Fitting Neural Network/Layer 1/IW{1,1} ==
  "pd{1,1}" : Inport  PortDimensions=2
      mask Display: e = 0.06;c1 = [120 230 180]/255;c2 = ([120 230 180]+0)/(256+128);c3 = ([120 230 180]+128)/(256+128);patch([0 1 1 0],[0 0 1 1],c1);patch([0 1 1 1-e 1-e 0+e],[0 0 1 1-e 0+e 0+e],c2);patch([0 0 1 1-e 0+e 0+e],[0 1 1 1-e 1-e 0+e],c3);plot([0 1 1 0 0],[0 0 1 1 0]);
  "IW{1,1}(1,:)'" : Constant  Value=[-3.1549215803620769;-3.2643744480250154]
      mask Display: e = 0.06;c1 = [120 150 230]/255;c2 = ([120 150 230]+0)/383;c3 = ([120 150 230]+128)/383;patch([0 1 1 0],[0 0 1 1],c1);patch([0 1 1 1-e 1-e 0+e],[0 0 1 1-e 0+e 0+e],c2);patch([0 0 1 1-e 0+e 0+e],[0 1 1 1-e 1-e 0+e],c3);plot([0 1 1 0 0],[0 0 1 1 0]);disp('Weights');
  "IW{1,1}(10,:)'" : Constant  Value=[4.3215386797726278;0.99216339136282483]
      mask Display: e = 0.06;c1 = [120 150 230]/255;c2 = ([120 150 230]+0)/383;c3 = ([120 150 230]+128)/383;patch([0 1 1 0],[0 0 1 1],c1);patch([0 1 1 1-e 1-e 0+e],[0 0 1 1-e 0+e 0+e],c2);patch([0 0 1 1-e 0+e 0+e],[0 1 1 1-e 1-e 0+e],c3);plot([0 1 1 0 0],[0 0 1 1 0]);disp('Weights');
  "IW{1,1}(2,:)'" : Constant  Value=[0.23159732733208307;4.3157665777225613]
      mask Display: e = 0.06;c1 = [120 150 230]/255;c2 = ([120 150 230]+0)/383;c3 = ([120 150 230]+128)/383;patch([0 1 1 0],[0 0 1 1],c1);patch([0 1 1 1-e 1-e 0+e],[0 0 1 1-e 0+e 0+e],c2);patch([0 0 1 1-e 0+e 0+e],[0 1 1 1-e 1-e 0+e],c3);plot([0 1 1 0 0],[0 0 1 1 0]);disp('Weights');
  "IW{1,1}(3,:)'" : Constant  Value=[3.5420645061139471;-3.668117065884676]
      mask Display: e = 0.06;c1 = [120 150 230]/255;c2 = ([120 150 230]+0)/383;c3 = ([120 150 230]+128)/383;patch([0 1 1 0],[0 0 1 1],c1);patch([0 1 1 1-e 1-e 0+e],[0 0 1 1-e 0+e 0+e],c2);patch([0 0 1 1-e 0+e 0+e],[0 1 1 1-e 1-e 0+e],c3);plot([0 1 1 0 0],[0 0 1 1 0]);disp('Weights');
  "IW{1,1}(4,:)'" : Constant  Value=[-2.4035631287998678;-3.9100394754890733]
      mask Display: e = 0.06;c1 = [120 150 230]/255;c2 = ([120 150 230]+0)/383;c3 = ([120 150 230]+128)/383;patch([0 1 1 0],[0 0 1 1],c1);patch([0 1 1 1-e 1-e 0+e],[0 0 1 1-e 0+e 0+e],c2);patch([0 0 1 1-e 0+e 0+e],[0 1 1 1-e 1-e 0+e],c3);plot([0 1 1 0 0],[0 0 1 1 0]);disp('Weights');
  "IW{1,1}(5,:)'" : Constant  Value=[4.0774515809679546;1.834066988323666]
      mask Display: e = 0.06;c1 = [120 150 230]/255;c2 = ([120 150 230]+0)/383;c3 = ([120 150 230]+128)/383;patch([0 1 1 0],[0 0 1 1],c1);patch([0 1 1 1-e 1-e 0+e],[0 0 1 1-e 0+e 0+e],c2);patch([0 0 1 1-e 0+e 0+e],[0 1 1 1-e 1-e 0+e],c3);plot([0 1 1 0 0],[0 0 1 1 0]);disp('Weights');
  "IW{1,1}(6,:)'" : Constant  Value=[-1.881341446481233;-3.9804518155051025]
      mask Display: e = 0.06;c1 = [120 150 230]/255;c2 = ([120 150 230]+0)/383;c3 = ([120 150 230]+128)/383;patch([0 1 1 0],[0 0 1 1],c1);patch([0 1 1 1-e 1-e 0+e],[0 0 1 1-e 0+e 0+e],c2);patch([0 0 1 1-e 0+e 0+e],[0 1 1 1-e 1-e 0+e],c3);plot([0 1 1 0 0],[0 0 1 1 0]);disp('Weights');
  "IW{1,1}(7,:)'" : Constant  Value=[1.1949505190782121;-4.2927822654522396]
      mask Display: e = 0.06;c1 = [120 150 230]/255;c2 = ([120 150 230]+0)/383;c3 = ([120 150 230]+128)/383;patch([0 1 1 0],[0 0 1 1],c1);patch([0 1 1 1-e 1-e 0+e],[0 0 1 1-e 0+e 0+e],c2);patch([0 0 1 1-e 0+e 0+e],[0 1 1 1-e 1-e 0+e],c3);plot([0 1 1 0 0],[0 0 1 1 0]);disp('Weights');
  "IW{1,1}(8,:)'" : Constant  Value=[3.7823096605965238;2.3006830791871233]
      mask Display: e = 0.06;c1 = [120 150 230]/255;c2 = ([120 150 230]+0)/383;c3 = ([120 150 230]+128)/383;patch([0 1 1 0],[0 0 1 1],c1);patch([0 1 1 1-e 1-e 0+e],[0 0 1 1-e 0+e 0+e],c2);patch([0 0 1 1-e 0+e 0+e],[0 1 1 1-e 1-e 0+e],c3);plot([0 1 1 0 0],[0 0 1 1 0]);disp('Weights');
  "IW{1,1}(9,:)'" : Constant  Value=[3.0604426851434487;-3.1993045631098105]
      mask Display: e = 0.06;c1 = [120 150 230]/255;c2 = ([120 150 230]+0)/383;c3 = ([120 150 230]+128)/383;patch([0 1 1 0],[0 0 1 1],c1);patch([0 1 1 1-e 1-e 0+e],[0 0 1 1-e 0+e 0+e],c2);patch([0 0 1 1-e 0+e 0+e],[0 1 1 1-e 1-e 0+e],c3);plot([0 1 1 0 0],[0 0 1 1 0]);disp('Weights');
  Mux : Mux  Inputs=10
      mask Display: e = 0.06;c1 = [120 150 230]/255;c2 = ([120 150 230]+0)/383;c3 = ([120 150 230]+128)/383;patch([0 1 1 0],[0 0 1 1],c1);patch([0 1 1 1-e 1-e 0+e],[0 0 1 1-e 0+e 0+e],c2);patch([0 0 1 1-e 0+e 0+e],[0 1 1 1-e 1-e 0+e],c3);plot([0 1 1 0 0],[0 0 1 1 0]);disp('Mux');
  dotprod{1..10} (10 alike) : neural/Weight Functions/dotprod
  "iz{1,1}" : Outport
      mask Display: e = 0.06;c1 = [120 230 180]/255;c2 = ([120 230 180]+0)/(256+128);c3 = ([120 230 180]+128)/(256+128);patch([0 1 1 0],[0 0 1 1],c1);patch([0 1 1 1-e 1-e 0+e],[0 0 1 1-e 0+e 0+e],c2);patch([0 0 1 1-e 0+e 0+e],[0 1 1 1-e 1-e 0+e],c3);plot([0 1 1 0 0],[0 0 1 1 0]);
  wires:
  Mux/1 -> "iz{1,1}"/1
  dotprod10/1 -> Mux/10
  "IW{1,1}(10,:)'"/1 -> dotprod10/1
  dotprod9/1 -> Mux/9
  "IW{1,1}(9,:)'"/1 -> dotprod9/1
  dotprod8/1 -> Mux/8
  "IW{1,1}(8,:)'"/1 -> dotprod8/1
  dotprod7/1 -> Mux/7
  "IW{1,1}(7,:)'"/1 -> dotprod7/1
  dotprod6/1 -> Mux/6
  "IW{1,1}(6,:)'"/1 -> dotprod6/1
  dotprod5/1 -> Mux/5
  "IW{1,1}(5,:)'"/1 -> dotprod5/1
  dotprod4/1 -> Mux/4
  "IW{1,1}(4,:)'"/1 -> dotprod4/1
  dotprod3/1 -> Mux/3
  "IW{1,1}(3,:)'"/1 -> dotprod3/1
  dotprod2/1 -> Mux/2
  "IW{1,1}(2,:)'"/1 -> dotprod2/1
  dotprod1/1 -> Mux/1
  "pd{1,1}"/1 -> dotprod10/2, dotprod9/2, dotprod8/2, dotprod7/2, dotprod6/2, dotprod5/2, dotprod4/2, dotprod3/2, dotprod2/2, dotprod1/2
  "IW{1,1}(1,:)'"/1 -> dotprod1/1

== system PV_SYSTEM_WITH_VARIOUS_MPPT/MATLAB//SIMULINK  BLOCK/ANN based MPPT/Function Fitting Neural Network/Layer 2/Delays 1 ==
  "p{2}" : Inport  PortDimensions=10
      mask Display: e = 0.06;c1 = [120 230 180]/255;c2 = ([120 230 180]+0)/(256+128);c3 = ([120 230 180]+128)/(256+128);patch([0 1 1 0],[0 0 1 1],c1);patch([0 1 1 1-e 1-e 0+e],[0 0 1 1-e 0+e 0+e],c2);patch([0 0 1 1-e 0+e 0+e],[0 1 1 1-e 1-e 0+e],c3);plot([0 1 1 0 0],[0 0 1 1 0]);
  mux : Mux  Inputs=1
      mask Display: e = 0.06;c1 = [120 150 230]/255;c2 = ([120 150 230]+0)/383;c3 = ([120 150 230]+128)/383;patch([0 1 1 0],[0 0 1 1],c1);patch([0 1 1 1-e 1-e 0+e],[0 0 1 1-e 0+e 0+e],c2);patch([0 0 1 1-e 0+e 0+e],[0 1 1 1-e 1-e 0+e],c3);plot([0 1 1 0 0],[0 0 1 1 0]);disp('Mux')
  "pd{2,1}" : Outport
      mask Display: e = 0.06;c1 = [120 230 180]/255;c2 = ([120 230 180]+0)/(256+128);c3 = ([120 230 180]+128)/(256+128);patch([0 1 1 0],[0 0 1 1],c1);patch([0 1 1 1-e 1-e 0+e],[0 0 1 1-e 0+e 0+e],c2);patch([0 0 1 1-e 0+e 0+e],[0 1 1 1-e 1-e 0+e],c3);plot([0 1 1 0 0],[0 0 1 1 0]);
  wires:
  mux/1 -> "pd{2,1}"/1
  "p{2}"/1 -> mux/1

== system PV_SYSTEM_WITH_VARIOUS_MPPT/MATLAB//SIMULINK  BLOCK/ANN based MPPT/Function Fitting Neural Network/Layer 2/LW{2,1} ==
  "ad{2,1}" : Inport  PortDimensions=10
      mask Display: e = 0.06;c1 = [120 230 180]/255;c2 = ([120 230 180]+0)/(256+128);c3 = ([120 230 180]+128)/(256+128);patch([0 1 1 0],[0 0 1 1],c1);patch([0 1 1 1-e 1-e 0+e],[0 0 1 1-e 0+e 0+e],c2);patch([0 0 1 1-e 0+e 0+e],[0 1 1 1-e 1-e 0+e],c3);plot([0 1 1 0 0],[0 0 1 1 0]);
  "IW{2,1}(1,:)'" : Constant  Value=[-0.47493517034765337;-0.41876239213672239;2.3962932035510089;-1.6611049994323526;-1.3129808401076486;-0.072751763885582382;-0.68753464914676288;-0.36606316852898096;0.45441754060086159;-0.26447547932800886]
      mask Display: e = 0.06;c1 = [120 150 230]/255;c2 = ([120 150 230]+0)/383;c3 = ([120 150 230]+128)/383;patch([0 1 1 0],[0 0 1 1],c1);patch([0 1 1 1-e 1-e 0+e],[0 0 1 1-e 0+e 0+e],c2);patch([0 0 1 1-e 0+e 0+e],[0 1 1 1-e 1-e 0+e],c3);plot([0 1 1 0 0],[0 0 1 1 0]);disp('weights');
  Mux : Mux  Inputs=1
      mask Display: e = 0.06;c1 = [120 150 230]/255;c2 = ([120 150 230]+0)/383;c3 = ([120 150 230]+128)/383;patch([0 1 1 0],[0 0 1 1],c1);patch([0 1 1 1-e 1-e 0+e],[0 0 1 1-e 0+e 0+e],c2);patch([0 0 1 1-e 0+e 0+e],[0 1 1 1-e 1-e 0+e],c3);plot([0 1 1 0 0],[0 0 1 1 0]);disp('Mux');
  dotprod1 : neural/Weight Functions/dotprod
  "lz{2,1}" : Outport
      mask Display: e = 0.06;c1 = [120 230 180]/255;c2 = ([120 230 180]+0)/(256+128);c3 = ([120 230 180]+128)/(256+128);patch([0 1 1 0],[0 0 1 1],c1);patch([0 1 1 1-e 1-e 0+e],[0 0 1 1-e 0+e 0+e],c2);patch([0 0 1 1-e 0+e 0+e],[0 1 1 1-e 1-e 0+e],c3);plot([0 1 1 0 0],[0 0 1 1 0]);
  wires:
  Mux/1 -> "lz{2,1}"/1
  dotprod1/1 -> Mux/1
  "ad{2,1}"/1 -> dotprod1/2
  "IW{2,1}(1,:)'"/1 -> dotprod1/1

== matlab function PV_SYSTEM_WITH_VARIOUS_MPPT/MATLAB//SIMULINK  BLOCK/X-Y Plotter/X-Y Animated Plotter ==
  data: x input; y input; set input
% Razman Ayop
% Created on 7 Nov 19

function xyplotanimate(x,y,set)

mem=10e3;            %Memory storage for the tail of the plot

%% Assign setting parameters
N=set(1);
xmin=set(2);
xmax=set(3);
ymin=set(4);
ymax=set(5);

%% System setting
persistent st;              % Allow parameter to maintain inside function (memory)
coder.extrinsic('delete')   % Allow delete function to be used in the function

%% Initiate Plotter
if isempty(st)
close all;
figure('Name','P-V Plotter','NumberTitle','off');
% Setting up plotter
axis([xmin xmax ymin ymax]);
grid on;
hold on;
xlabel('PV Voltage, V_p_v (V)');
ylabel('PV Power, P_p_v (W)');
% Setting up memory
st.i=1;   % Location of plot creation
st.j=1;   % Location of plot deletion
st.k=0;   % Switching on plot deletion
st.h=zeros(1,mem);  % Memory storage

%% Running Plotter
else
    st.h(st.i)=plot(x,y,'kx');  % Plot graph
    st.i=st.i+1;
    if st.i>N                   % Location for plot creation full
        st.i=1;
        st.k=1;
    end
    if st.k==1                  % Initiate delete older data
        delete(st.h(st.j));
        st.j=st.j+1;
    end
    if st.j>N                   % Reset location for plot deletion
        st.j=1;
    end
end
